simulink model "control_logic"  (R2025b)
settings: Solver=FixedStepDiscrete  StartTime=0.0  StopTime=10.0  FixedStep=0.1  RelTol=1e-3
settings Model: Creator=R  LastModifiedBy=R

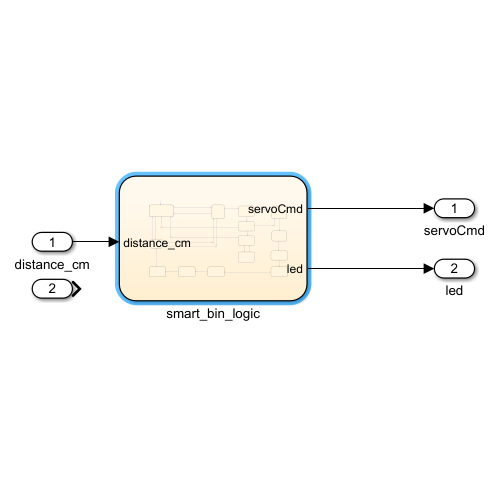
[thumbnail: Simulink's stored preview of the top-level diagram]
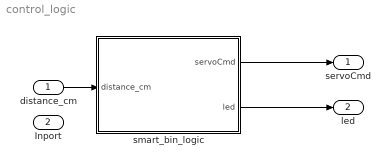
== system control_logic ==
  distance_cm : Inport
  Inport : Inport  Port=2
  smart_bin_logic : Stateflow chart  TreatAsAtomicUnit=on
  servoCmd : Outport
  led : Outport  Port=2
  wires:
  distance_cm/1 -> smart_bin_logic/1(distance_cm)
  smart_bin_logic/1(servoCmd) -> servoCmd/1
  smart_bin_logic/2(led) -> led/1

== stateflow chart control_logic/smart_bin_logic ==
  state CLOSED_IDLE
    entry:
    servoCmd = 0;
    led = 0;
  state REQUEST_WAIT
    entry:
    servoCmd = 0;
    led = 0;
  state HALF_OPEN_BLINK
    entry:
    servoCmd = 90;
    led = 1;
  state OPEN_BLINK
    entry:
    servoCmd = 180;
    led = 1;
  state HALF_OPEN_WAIT
    entry:
    servoCmd = 90;
    led = 0;
  state OPEN_WAIT
    entry:
    servoCmd = 180;
    led = 0;
  state TIMEOUT_BLINK_ON
    entry:
    servoCmd = 0;
    led = 1;
  state TOO_CLOSE
    entry:
    servoCmd = 0;
    led = 1;
  state CLOSE_BLINK1_ON
    entry:
    servoCmd = 0;
    led = 1;
  state TIMEOUT_BLINK_OFF
    entry:
    servoCmd = 0;
    led = 0;
  state COOLDOWN
    entry:
    servoCmd = 0;
    led = 0;
  state CLOSE_BLINK2_OFF
    entry:
    servoCmd = 0;
    led = 0;
  state CLOSE_BLINK2_ON
    entry:
    servoCmd = 0;
    led = 1;
  state CLOSE_BLINK1_OFF
    entry:
    servoCmd = 0;
    led = 0;
  (default) -> CLOSED_IDLE
  CLOSED_IDLE -> REQUEST_WAIT [order 2] : [distance_cm > 0.5 && distance_cm <= 2.5]
  REQUEST_WAIT -> HALF_OPEN_BLINK [order 3] : [after(5, sec)]
  HALF_OPEN_BLINK -> OPEN_BLINK [order 2] : [distance_cm <= 1]
  REQUEST_WAIT -> CLOSED_IDLE [order 1] : [distance_cm > 2.5]
  HALF_OPEN_BLINK -> HALF_OPEN_WAIT [order 1] : [after(1, sec)]
  TOO_CLOSE -> CLOSED_IDLE [order 2] : [distance_cm > 2.5]
  CLOSED_IDLE -> TOO_CLOSE [order 1] : [distance_cm <= 0.5]
  (junction 55) -> CLOSED_IDLE
  (junction 53) -> CLOSED_IDLE
  (junction 49) -> REQUEST_WAIT
  REQUEST_WAIT -> (junction 51) [order 2] : [distance_cm <= 0.5]
  (junction 59) -> OPEN_BLINK
  OPEN_BLINK -> OPEN_WAIT : [after(1, sec)]
  HALF_OPEN_WAIT -> (junction 59) [order 1] : [distance_cm <= 1]
  HALF_OPEN_WAIT -> (junction 55) [order 3] : [distance_cm > 2.5]
  HALF_OPEN_WAIT -> TIMEOUT_BLINK_ON [order 2] : [after(9, sec)]
  TIMEOUT_BLINK_ON -> (junction 53) [order 1] : [distance_cm > 2.5]
  OPEN_WAIT -> CLOSE_BLINK1_ON : [after(9, sec)]
  TOO_CLOSE -> (junction 49) [order 1] : [distance_cm > 0.5 && distance_cm <= 2.5]
  TIMEOUT_BLINK_ON -> TIMEOUT_BLINK_OFF [order 2] : [after(1, sec)]
  TIMEOUT_BLINK_OFF -> TIMEOUT_BLINK_ON : [after(1, sec)]
  (junction 51) -> TOO_CLOSE
  COOLDOWN -> TOO_CLOSE : [after(30, sec)]
  CLOSE_BLINK1_ON -> CLOSE_BLINK1_OFF : [after(1, sec)]
  CLOSE_BLINK2_ON -> CLOSE_BLINK2_OFF : [after(1, sec)]
  CLOSE_BLINK2_OFF -> COOLDOWN : [after(1, sec)]
  CLOSE_BLINK1_OFF -> CLOSE_BLINK2_ON : [after(1, sec)]
  data: distance_cm input; servoCmd output; led output
